simulink model "Quadri_Victor_combination_PID_R2025a_CE"  (R2025a)
settings: Solver=FixedStepDiscrete  StartTime=0.0  StopTime=quad_t_stop  FixedStep=pid_dt  RelTol=1e-3  EnableMultiTasking=on
InitFcn:
  | run(fullfile(fileparts(fileparts(get_param(bdroot,'FileName'))),'params','victor_pid_params.m'))
undefined symbols (not defined in the file): pid_dt, quad_param_vec, quad_x0
settings Model: ExtModeTrigDuration=10000  Creator=gandhico  LastModifiedBy=gandhico
settings SolverCC: AlgebraicLoopSolver=TrustRegion  PositivePriorityOrder=on
settings DataIOCC: ReturnWorkspaceOutputs=off
settings DebuggingCC: UnconnectedInputMsg=warning  UnconnectedOutputMsg=warning  UnconnectedLineMsg=warning  ArithmeticOperatorsInVariantConditions=warning
settings ModelReferenceCC: EnableRefExpFcnMdlSchedulingChecks=on
settings SFSimCC: SimUseLocalCustomCode=off  CustomCodeUndefinedFunction=UseInterfaceOnly
settings RTWCC: RTWUseLocalCustomCode=off  Toolchain=QUARC win64 | nmake (64-bit Windows)  BuildConfiguration=Faster Runs  GPUComputeCapability=3.5
settings CodeAppCC: StateflowObjectComments=on
settings ConfigComp: CovMetricSettings=dswe

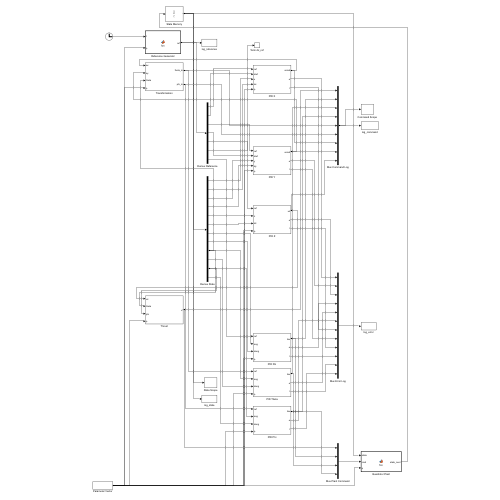
[thumbnail: Simulink's stored preview of the top-level diagram]
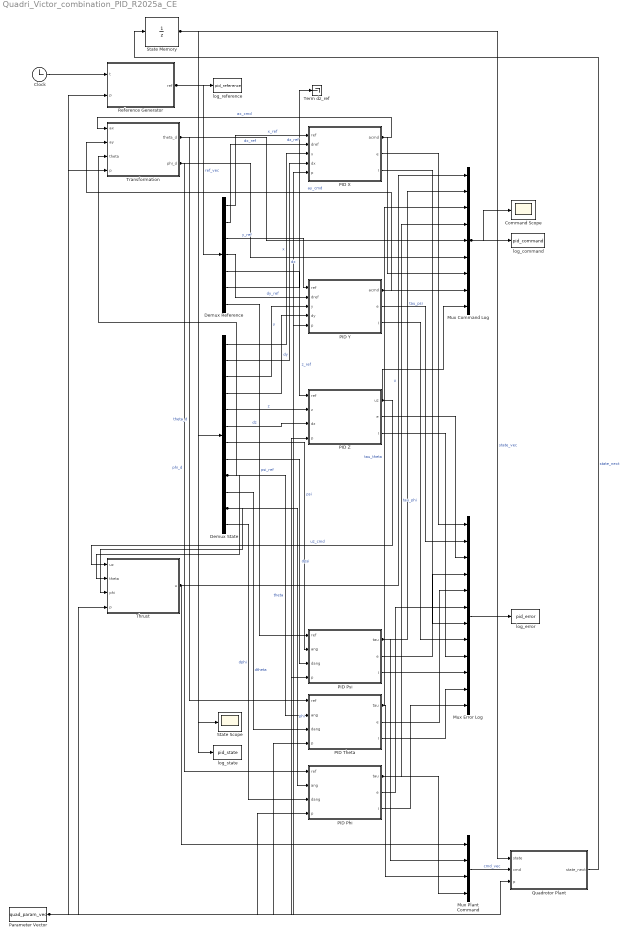
== system Quadri_Victor_combination_PID_R2025a_CE ==
  Clock : Clock
  Command Scope : Scope
  Demux Reference : Demux  Outputs=7
  Demux State : Demux  Outputs=12
  Mux Command Log : Mux  Inputs=9
  Mux Error Log : Mux  Inputs=12
  Mux Plant Command : Mux
  PID Phi : Subsystem
  PID Psi : Subsystem
  PID Theta : Subsystem
  PID X : Subsystem
  PID Y : Subsystem
  PID Z : Subsystem
  Parameter Vector : Constant  Value=quad_param_vec
  Quadrotor Plant : MATLAB Function  TreatAsAtomicUnit=on
  Reference Generator : MATLAB Function  TreatAsAtomicUnit=on
  State Memory : UnitDelay  InitialCondition=quad_x0  SampleTime=pid_dt  HasFrameUpgradeWarning=on
  State Scope : Scope
  Term dz_ref : Terminator
  Thrust : Subsystem
  Transformation : Subsystem
  log_command : ToWorkspace  VariableName=pid_command  SaveFormat=Structure With Time  SampleTime=-1
  log_error : ToWorkspace  VariableName=pid_error  SaveFormat=Structure With Time  SampleTime=-1
  log_reference : ToWorkspace  VariableName=pid_reference  SaveFormat=Structure With Time  SampleTime=-1
  log_state : ToWorkspace  VariableName=pid_state  SaveFormat=Structure With Time  SampleTime=-1
  wires:
  Clock/1 -> Reference Generator/1(t)
  Thrust/1(u) -> Mux Plant Command/1, Mux Command Log/1  "u"
  Transformation/2(phi_d) -> Mux Command Log/6, PID Phi/1(ref)  "phi_d"
  Demux Reference/3 -> PID Y/1(ref)  "y_ref"
  Parameter Vector/1 -> PID X/5(p), PID Y/5(p), PID Psi/4(p), PID Theta/4(p), PID Phi/4(p), PID Z/4(p), Quadrotor Plant/3(p), Reference Generator/2(p), Thrust/4(p), Transformation/4(p)
  Demux Reference/6 -> Term dz_ref/1  "dz_ref"
  State Memory/1 -> Quadrotor Plant/1(state), Demux State/1, log_state/1, State Scope/1  "state_vec"
  Mux Plant Command/1 -> Quadrotor Plant/2(cmd)  "cmd_vec"
  Reference Generator/1(ref) -> Demux Reference/1, log_reference/1  "ref_vec"
  Transformation/1(theta_d) -> PID Theta/1(ref), Mux Command Log/5  "theta_d"
  Demux State/9 -> Transformation/3(theta), Thrust/2(theta), PID Theta/2(ang)  "theta"
  Demux State/5 -> PID Z/2(z)  "z"
  Demux Reference/1 -> PID X/1(ref)  "x_ref"
  PID Theta/2(e) -> Mux Error Log/5
  PID Y/3(I) -> Mux Error Log/8
  Demux Reference/2 -> PID X/2(dref)  "dx_ref"
  Demux Reference/4 -> PID Y/2(dref)  "dy_ref"
  Demux Reference/5 -> PID Z/1(ref)  "z_ref"
  Demux Reference/7 -> PID Psi/1(ref)  "psi_ref"
  PID Theta/1(tau) -> Mux Command Log/3, Mux Plant Command/3  "tau_theta"
  Demux State/4 -> PID Y/4(dy)  "dy"
  Demux State/1 -> PID X/3(x)  "x"
  Demux State/2 -> PID X/4(dx)  "dx"
  Demux State/3 -> PID Y/3(y)  "y"
  Mux Error Log/1 -> log_error/1
  Demux State/6 -> PID Z/3(dz)  "dz"
  Demux State/7 -> PID Psi/2(ang)  "psi"
  Demux State/8 -> PID Psi/3(dang)  "dpsi"
  PID Phi/3(I) -> Mux Error Log/12
  PID X/1(acmd) -> Mux Command Log/7, Transformation/1(ax)  "ax_cmd"
  Demux State/10 -> PID Theta/3(dang)  "dtheta"
  Demux State/11 -> Thrust/3(phi), PID Phi/2(ang)  "phi"
  PID Phi/2(e) -> Mux Error Log/6
  Demux State/12 -> PID Phi/3(dang)  "dphi"
  PID X/2(e) -> Mux Error Log/1
  PID X/3(I) -> Mux Error Log/7
  PID Y/1(acmd) -> Transformation/2(ay), Mux Command Log/8  "ay_cmd"
  PID Y/2(e) -> Mux Error Log/2
  PID Z/1(uz) -> Mux Command Log/9, Thrust/1(uz)  "uz_cmd"
  PID Z/2(e) -> Mux Error Log/3
  PID Z/3(I) -> Mux Error Log/9
  PID Psi/1(tau) -> Mux Plant Command/2, Mux Command Log/2  "tau_psi"
  PID Psi/2(e) -> Mux Error Log/4
  PID Psi/3(I) -> Mux Error Log/10
  PID Theta/3(I) -> Mux Error Log/11
  PID Phi/1(tau) -> Mux Plant Command/4, Mux Command Log/4  "tau_phi"
  Mux Command Log/1 -> log_command/1, Command Scope/1
  Quadrotor Plant/1(state_next) -> State Memory/1  "state_next"

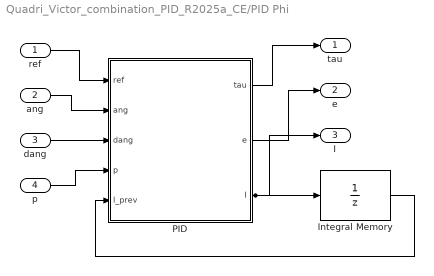
== system Quadri_Victor_combination_PID_R2025a_CE/PID Phi ==
  ref : Inport
  ang : Inport  Port=2
  dang : Inport  Port=3
  p : Inport  Port=4
  Integral Memory : UnitDelay  SampleTime=pid_dt  HasFrameUpgradeWarning=on
  PID : MATLAB Function  TreatAsAtomicUnit=on
  tau : Outport
  e : Outport  Port=2
  I : Outport  Port=3
  wires:
  ang/1 -> PID/2(ang)
  ref/1 -> PID/1(ref)
  dang/1 -> PID/3(dang)
  Integral Memory/1 -> PID/5(I_prev)
  PID/2(e) -> e/1
  p/1 -> PID/4(p)
  PID/3(I) -> I/1, Integral Memory/1
  PID/1(tau) -> tau/1

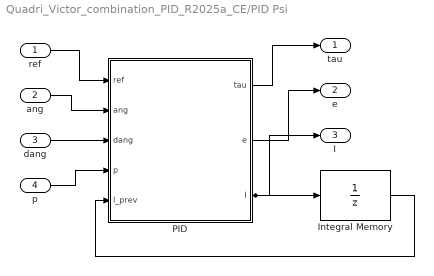
== system Quadri_Victor_combination_PID_R2025a_CE/PID Psi ==
  ref : Inport
  ang : Inport  Port=2
  dang : Inport  Port=3
  p : Inport  Port=4
  Integral Memory : UnitDelay  SampleTime=pid_dt  HasFrameUpgradeWarning=on
  PID : MATLAB Function  TreatAsAtomicUnit=on
  tau : Outport
  e : Outport  Port=2
  I : Outport  Port=3
  wires:
  PID/1(tau) -> tau/1
  ref/1 -> PID/1(ref)
  ang/1 -> PID/2(ang)
  PID/3(I) -> I/1, Integral Memory/1
  dang/1 -> PID/3(dang)
  p/1 -> PID/4(p)
  Integral Memory/1 -> PID/5(I_prev)
  PID/2(e) -> e/1

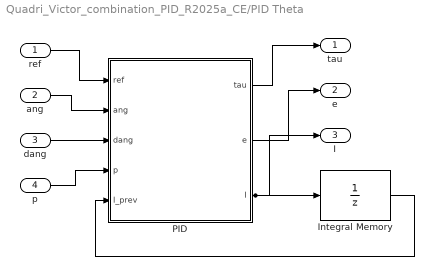
== system Quadri_Victor_combination_PID_R2025a_CE/PID Theta ==
  ref : Inport
  ang : Inport  Port=2
  dang : Inport  Port=3
  p : Inport  Port=4
  Integral Memory : UnitDelay  SampleTime=pid_dt  HasFrameUpgradeWarning=on
  PID : MATLAB Function  TreatAsAtomicUnit=on
  tau : Outport
  e : Outport  Port=2
  I : Outport  Port=3
  wires:
  PID/3(I) -> I/1, Integral Memory/1
  ang/1 -> PID/2(ang)
  ref/1 -> PID/1(ref)
  Integral Memory/1 -> PID/5(I_prev)
  dang/1 -> PID/3(dang)
  p/1 -> PID/4(p)
  PID/1(tau) -> tau/1
  PID/2(e) -> e/1

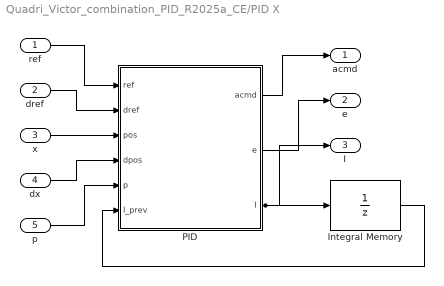
== system Quadri_Victor_combination_PID_R2025a_CE/PID X ==
  ref : Inport
  dref : Inport  Port=2
  x : Inport  Port=3
  dx : Inport  Port=4
  p : Inport  Port=5
  Integral Memory : UnitDelay  SampleTime=pid_dt  HasFrameUpgradeWarning=on
  PID : MATLAB Function  TreatAsAtomicUnit=on
  acmd : Outport
  e : Outport  Port=2
  I : Outport  Port=3
  wires:
  x/1 -> PID/3(pos)
  PID/1(acmd) -> acmd/1
  ref/1 -> PID/1(ref)
  dref/1 -> PID/2(dref)
  dx/1 -> PID/4(dpos)
  PID/3(I) -> I/1, Integral Memory/1
  p/1 -> PID/5(p)
  PID/2(e) -> e/1
  Integral Memory/1 -> PID/6(I_prev)

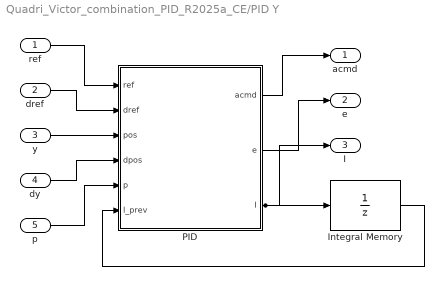
== system Quadri_Victor_combination_PID_R2025a_CE/PID Y ==
  ref : Inport
  dref : Inport  Port=2
  y : Inport  Port=3
  dy : Inport  Port=4
  p : Inport  Port=5
  Integral Memory : UnitDelay  SampleTime=pid_dt  HasFrameUpgradeWarning=on
  PID : MATLAB Function  TreatAsAtomicUnit=on
  acmd : Outport
  e : Outport  Port=2
  I : Outport  Port=3
  wires:
  PID/1(acmd) -> acmd/1
  ref/1 -> PID/1(ref)
  PID/3(I) -> I/1, Integral Memory/1
  dref/1 -> PID/2(dref)
  y/1 -> PID/3(pos)
  PID/2(e) -> e/1
  dy/1 -> PID/4(dpos)
  p/1 -> PID/5(p)
  Integral Memory/1 -> PID/6(I_prev)

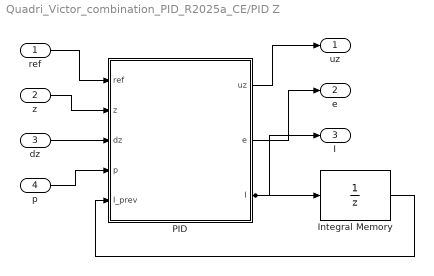
== system Quadri_Victor_combination_PID_R2025a_CE/PID Z ==
  ref : Inport
  z : Inport  Port=2
  dz : Inport  Port=3
  p : Inport  Port=4
  Integral Memory : UnitDelay  SampleTime=pid_dt  HasFrameUpgradeWarning=on
  PID : MATLAB Function  TreatAsAtomicUnit=on
  uz : Outport
  e : Outport  Port=2
  I : Outport  Port=3
  wires:
  z/1 -> PID/2(z)
  ref/1 -> PID/1(ref)
  PID/2(e) -> e/1
  dz/1 -> PID/3(dz)
  p/1 -> PID/4(p)
  PID/1(uz) -> uz/1
  PID/3(I) -> I/1, Integral Memory/1
  Integral Memory/1 -> PID/5(I_prev)

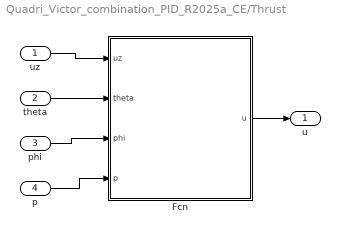
== system Quadri_Victor_combination_PID_R2025a_CE/Thrust ==
  uz : Inport
  theta : Inport  Port=2
  phi : Inport  Port=3
  p : Inport  Port=4
  Fcn : MATLAB Function  TreatAsAtomicUnit=on
  u : Outport
  wires:
  Fcn/1(u) -> u/1
  phi/1 -> Fcn/3(phi)
  uz/1 -> Fcn/1(uz)
  p/1 -> Fcn/4(p)
  theta/1 -> Fcn/2(theta)

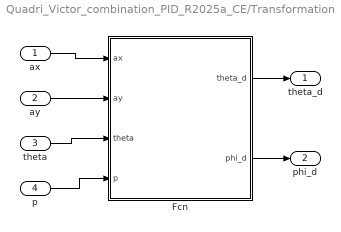
== system Quadri_Victor_combination_PID_R2025a_CE/Transformation ==
  ax : Inport
  ay : Inport  Port=2
  theta : Inport  Port=3
  p : Inport  Port=4
  Fcn : MATLAB Function  TreatAsAtomicUnit=on
  theta_d : Outport
  phi_d : Outport  Port=2
  wires:
  ay/1 -> Fcn/2(ay)
  ax/1 -> Fcn/1(ax)
  theta/1 -> Fcn/3(theta)
  p/1 -> Fcn/4(p)
  Fcn/1(theta_d) -> theta_d/1
  Fcn/2(phi_d) -> phi_d/1

== matlab function Quadri_Victor_combination_PID_R2025a_CE/PID Phi/PID ==
  data: ref input; tau output; ang input; dang input; p input size=[36 1]; I_prev input; e output; I output
function [tau, e, I] = fcn(ref, ang, dang, p, I_prev)
%#codegen
dt = p(1);
kp = p(24); ki = p(25); kd = p(26); ilim = p(36); taulim = p(33);
e = ref - ang;
de = -dang;
I = min(max(I_prev + dt*e, -ilim), ilim);
tau = min(max(kp*e + ki*I + kd*de, -taulim), taulim);
end

== matlab function Quadri_Victor_combination_PID_R2025a_CE/Thrust/Fcn ==
  data: uz input; u output; theta input; phi input; p input size=[36 1]
function u = fcn(uz, theta, phi, p)
%#codegen
m = p(2); g = p(3); den_min = p(28); u_min = p(29); u_max = p(30);
u_unsat = (m*g + uz)/max(cos(theta)*cos(phi), den_min);
u = min(max(u_unsat, u_min), u_max);
end

== matlab function Quadri_Victor_combination_PID_R2025a_CE/Quadrotor Plant ==
  data: state input size=[12 1]; state_next output size=[12 1]; cmd input size=[4 1]; p input size=[36 1]
function state_next = fcn(state, cmd, p)
%#codegen
h = p(1);
k1 = dyn_quad(state, cmd, p);
k2 = dyn_quad(state + 0.5*h*k1, cmd, p);
k3 = dyn_quad(state + 0.5*h*k2, cmd, p);
k4 = dyn_quad(state + h*k3, cmd, p);
state_next = state + (h/6.0)*(k1 + 2.0*k2 + 2.0*k3 + k4);
end

function dX = dyn_quad(x, cmd, p)
m = p(2);
g = p(3);
u = cmd(1);
tau_psi = cmd(2);
tau_theta = cmd(3);
tau_phi = cmd(4);
psi = x(7); theta = x(9); phi = x(11);

dX = zeros(12,1);
dX(1) = x(2);
dX(2) = u*(sin(phi)*sin(psi) + cos(phi)*cos(psi)*sin(theta))/m;
dX(3) = x(4);
dX(4) = u*(cos(phi)*sin(theta)*sin(psi) - cos(psi)*sin(phi))/m;
dX(5) = x(6);
dX(6) = u*(cos(theta)*cos(phi))/m - g;
dX(7) = x(8);
dX(8) = tau_psi;
dX(9) = x(10);
dX(10) = tau_theta;
dX(11) = x(12);
dX(12) = tau_phi;
end

== matlab function Quadri_Victor_combination_PID_R2025a_CE/Reference Generator ==
  data: t input size=[1 1]; ref output size=[7 1]; p input size=[36 1]
function ref = fcn(t, p)
%#codegen
k = p(4);
z_amp = p(5);
x_amp = p(6);
y_amp = p(7);
psi_ref_value = p(8);

% --- Sigmoid trajectory mission ----------------------------------------
%   x_d(t) = x_amp / (1 + exp(-k*(t - 5)))                  center 5, no delay
%   z_d(t) = z_amp / (1 + exp(-k*(t - 4)))                  center 4, no delay
%   y_d(t) = 0                              for t <  y_delay
%          = y_amp / (1 + exp(-k*((t - y_delay) - 5)))      center 5, delayed
% Amplitudes (x_amp, y_amp, z_amp) and k come from params/victor_pid_params.m;
% the centers and the y-channel delay are defined here.
y_delay = 15.0;

[z_ref, dz_sigmoid] = sigmoid_ref(t, z_amp, k, 4.0);
[x_ref, dx_ref] = sigmoid_ref(t, x_amp, k, 5.0);
if t < y_delay
    y_ref = 0.0;
    dy_ref = 0.0;
else
    [y_ref, dy_ref] = sigmoid_ref(t - y_delay, y_amp, k, 5.0);
end

% The original Victor Fcn z controller damps measured dz only; it does not
% subtract dz_ref. Keep this channel zero to make that convention explicit.
dz_ref = 0.0;
psi_ref = psi_ref_value;
ref = [x_ref; dx_ref; y_ref; dy_ref; z_ref; dz_ref; psi_ref];
end

function [r, dr] = sigmoid_ref(t, amp, k, center)
q = exp(-k*(t - center));
den = 1.0 + q;
r = amp/den;
dr = amp*k*q/(den*den);
end

== matlab function Quadri_Victor_combination_PID_R2025a_CE/PID X/PID ==
  data: ref input; acmd output; dref input; pos input; dpos input; p input size=[36 1]; I_prev input; e output; I output
function [acmd, e, I] = fcn(ref, dref, pos, dpos, p, I_prev)
%#codegen
dt = p(1);
kp = p(12); ki = p(13); kd = p(14); ilim = p(34);
e = ref - pos;
de = dref - dpos;
I = min(max(I_prev + dt*e, -ilim), ilim);
acmd = kp*e + ki*I + kd*de;
end

== matlab function Quadri_Victor_combination_PID_R2025a_CE/PID Y/PID ==
  data: ref input; acmd output; dref input; pos input; dpos input; p input size=[36 1]; I_prev input; e output; I output
function [acmd, e, I] = fcn(ref, dref, pos, dpos, p, I_prev)
%#codegen
dt = p(1);
kp = p(15); ki = p(16); kd = p(17); ilim = p(34);
e = ref - pos;
de = dref - dpos;
I = min(max(I_prev + dt*e, -ilim), ilim);
acmd = kp*e + ki*I + kd*de;
end

== matlab function Quadri_Victor_combination_PID_R2025a_CE/PID Z/PID ==
  data: ref input; uz output; z input; dz input; p input size=[36 1]; I_prev input; e output; I output
function [uz, e, I] = fcn(ref, z, dz, p, I_prev)
%#codegen
dt = p(1);
kp = p(9); ki = p(10); kd = p(11); ilim = p(35);
e = ref - z;
de = -dz;
I = min(max(I_prev + dt*e, -ilim), ilim);
uz = kp*e + ki*I + kd*de;
end

== matlab function Quadri_Victor_combination_PID_R2025a_CE/Transformation/Fcn ==
  data: ax input; theta_d output; ay input; theta input; p input size=[36 1]; phi_d output
function [theta_d, phi_d] = fcn(ax, ay, theta, p)
%#codegen
g = p(3); tilt = p(27);
theta_d = min(max(atan2(ax, g), -tilt), tilt);
phi_d = min(max(atan2(-ay*cos(theta), g), -tilt), tilt);
end

== matlab function Quadri_Victor_combination_PID_R2025a_CE/PID Psi/PID ==
  data: ref input; tau output; ang input; dang input; p input size=[36 1]; I_prev input; e output; I output
function [tau, e, I] = fcn(ref, ang, dang, p, I_prev)
%#codegen
dt = p(1);
kp = p(18); ki = p(19); kd = p(20); ilim = p(36); taulim = p(31);
e = mod((ref - ang) + pi, 2*pi) - pi;
de = -dang;
I = min(max(I_prev + dt*e, -ilim), ilim);
tau = min(max(kp*e + ki*I + kd*de, -taulim), taulim);
end

== matlab function Quadri_Victor_combination_PID_R2025a_CE/PID Theta/PID ==
  data: ref input; tau output; ang input; dang input; p input size=[36 1]; I_prev input; e output; I output
function [tau, e, I] = fcn(ref, ang, dang, p, I_prev)
%#codegen
dt = p(1);
kp = p(21); ki = p(22); kd = p(23); ilim = p(36); taulim = p(32);
e = ref - ang;
de = -dang;
I = min(max(I_prev + dt*e, -ilim), ilim);
tau = min(max(kp*e + ki*I + kd*de, -taulim), taulim);
end
